simulink model "gantry_move_test"  (R2025b)
settings: Solver=FixedStepDiscrete  StartTime=0.0  StopTime=inf  FixedStep=0.05  RelTol=1e-3  EnableMultiTasking=on
libraries: raspberrypiBasiclib x4
settings Model: Creator=jeets  LastModifiedBy=jeets
settings SolverCC: PositivePriorityOrder=on
settings OptimizationCC: EnhancedBackFolding=on  PassReuseOutputArgsAs=Individual arguments  ZeroExternalMemoryAtStartup=off  ZeroInternalMemoryAtStartup=off  MaxStackSize=200000  OptimizeBlockOrder=speed  DifferentSizesBufferReuse=on  OptimizationCustomize=off  EfficientTunableParamExpr=on
settings DebuggingCC: ParameterTunabilityLossMsg=error
settings HardwareCC: ProdBitPerPointer=32.0  ProdBitPerSizeT=32.0  ProdBitPerPtrDiffT=32.0  ProdLargestAtomicInteger=Long  ProdLargestAtomicFloat=Double  ProdWordSize=32.0  ProdLongLongMode=on  ProdHWDeviceType=ARM Compatible->ARM Cortex-A (32-bit)
settings RTWCC: SystemTargetFile=ert.tlc  HardwareBoard=Raspberry Pi  TLCOptions="-aInlineSetEventsForThisBaseRateFcn=TLC_FALSE -aSuppressMultiTaskScheduler=TLC_FALSE  -aRateBasedStepFcn=0"  TemplateMakefile=ert_default_tmf  Toolchain=GNU GCC Embedded Linux  BuildConfiguration=Faster Runs  Description=Embedded Coder
settings CodeAppCC: ForceParamTrailComments=on  IgnoreCustomStorageClasses=off  OperatorAnnotations=on  SimulinkDataObjDesc=on  SFDataObjDesc=on  InsertBlockDesc=on
settings ERTTargetCC: ExtModeTransport=2.0  ExtModeStaticAlloc=on  ExtModeMexFile=ext_xcp  ExtModeIntrfLevel=Level2 - Open  InlinedParameterPlacement=Hierarchical  CodeReplacementLibrary=ARM Cortex-A CMSIS  SupportVariableSizeSignals=on

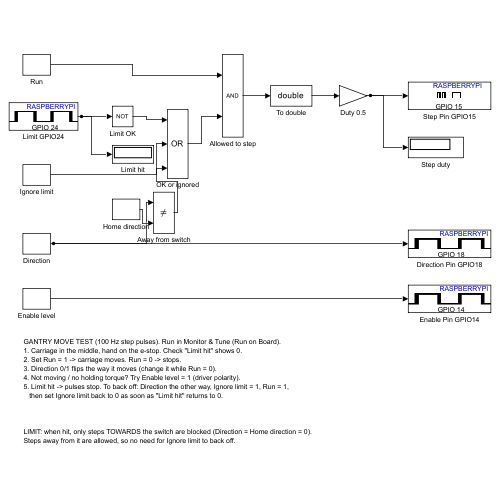
[thumbnail: Simulink's stored preview of the top-level diagram]
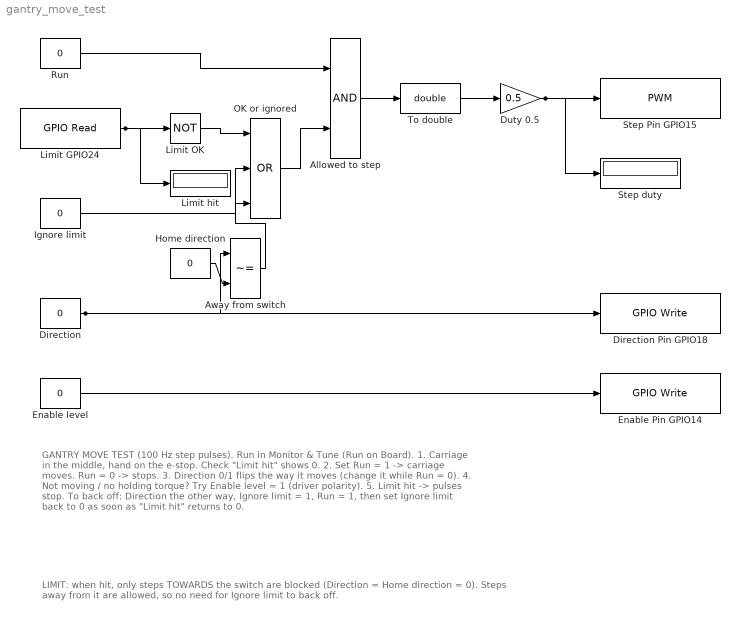
== system gantry_move_test ==
  note: GANTRY MOVE TEST (100 Hz step pulses). Run in Monitor & Tune (Run on Board).
      | 1. Carriage in the middle, hand on the e-stop. Check "Limit hit" shows 0.
      | 2. Set Run = 1 -> carriage moves. Run = 0 -> stops.
      | 3. Direction 0/1 flips the way it moves (change it while Run = 0).
      | 4. Not moving / no holding torque? Try Enable level = 1 (driver polarity).
      | 5. Limit hit -> pulses stop. To back off: Direction the other way, Ignore limit = 1, Run = 1,
      |    then set Ignore limit back to 0 as soon as "Limit hit" returns to 0.
  note: LIMIT: when hit, only steps TOWARDS the switch are blocked (Direction = Home direction = 0).
      | Steps away from it are allowed, so no need for Ignore limit to back off.
  Allowed to step : Logic  AllPortsSameDT=off  OutDataTypeStr=boolean
  Away from switch : RelationalOperator  Operator=~=  OutDataTypeStr=boolean  RndMeth=Simplest  InputSameDT=off
  Direction : Constant  Value=0  OutDataTypeStr=boolean
  Direction Pin GPIO18 : raspberrypiBasiclib/GPIO Write  BoardProperty=Pi 3 Model B+  gpio=18  blockPlatform=Raspberry Pi  PinNumber=17  board=[]  direction=[]
  Duty 0.5 : Gain  Gain=0.5
  Enable Pin GPIO14 : raspberrypiBasiclib/GPIO Write  BoardProperty=Pi 3 Model B+  gpio=14  blockPlatform=Raspberry Pi  PinNumber=17  board=[]  direction=[]
  Enable level : Constant  Value=0  OutDataTypeStr=boolean
  Home direction : Constant  Value=0
  Ignore limit : Constant  Value=0
  Limit GPIO24 : raspberrypiBasiclib/GPIO Read  BoardProperty=Pi 3 Model B+  gpio=24  SampleTime=0.05  blockPlatform=Raspberry Pi  PinNumber=4  board=[]  direction=[]  internalResistor=[]
  Limit OK : Logic  Operator=NOT  AllPortsSameDT=off  OutDataTypeStr=boolean
  Limit hit : Display
  OK or ignored : Logic  Operator=OR  Inputs=3  AllPortsSameDT=off  OutDataTypeStr=boolean
  Run : Constant  Value=0
  Step Pin GPIO15 : raspberrypiBasiclib/PWM  board=Pi 3 Model B+  Pin_=15  Frequency=100  blockPlatform=Raspberry Pi
  Step duty : Display
  To double : DataTypeConversion  OutDataTypeStr=double  SaturateOnIntegerOverflow=off  RndMeth=Floor
  wires:
  Limit GPIO24/1 -> Limit OK/1, Limit hit/1
  Limit OK/1 -> OK or ignored/1
  Ignore limit/1 -> OK or ignored/2
  Run/1 -> Allowed to step/1
  OK or ignored/1 -> Allowed to step/2
  Allowed to step/1 -> To double/1
  To double/1 -> Duty 0.5/1
  Duty 0.5/1 -> Step Pin GPIO15/1, Step duty/1
  Direction/1 -> Direction Pin GPIO18/1, Away from switch/1
  Enable level/1 -> Enable Pin GPIO14/1
  Home direction/1 -> Away from switch/2
  Away from switch/1 -> OK or ignored/3
